simulink model "hopping_daisy"  (R2026b)
settings: Solver=FixedStepDiscrete  StartTime=0  StopTime=10  FixedStep=1
values from neighbouring files (symbols this model uses):
  daisy_bitmap = <binary blob, 10705 chars, not shown>    [hopping_daisy_dd.sldd]
  DAISY_HEIGHT = 40.0    [hopping_daisy_dd.sldd]
  DAISY_WIDTH = 40.0    [hopping_daisy_dd.sldd]
  DAISY_X_START = 80.0    [hopping_daisy_dd.sldd]
  GAME_INIT = 1.0    [hopping_daisy_dd.sldd]
  GAME_STARTED = 2.0    [hopping_daisy_dd.sldd]
  GAME_STOPPED = 3.0    [hopping_daisy_dd.sldd]
  GROUND_BLUE = 64.0    [hopping_daisy_dd.sldd]
  GROUND_GREEN = 176.0    [hopping_daisy_dd.sldd]
  GROUND_RED = 48.0    [hopping_daisy_dd.sldd]
  GROUND_Y_START = 400.0    [hopping_daisy_dd.sldd]
  H_SYNC_END = 752.0    [hopping_daisy_dd.sldd]
  H_SYNC_START = 656.0    [hopping_daisy_dd.sldd]
  H_TOTAL = 800.0    [hopping_daisy_dd.sldd]
  H_VISIBLE = 640.0    [hopping_daisy_dd.sldd]
  obstacle_bitmap = <binary blob, 6837 chars, not shown>    [hopping_daisy_dd.sldd]
  OBSTACLE_HEIGHT = 40.0    [hopping_daisy_dd.sldd]
  OBSTACLE_WIDTH = 20.0    [hopping_daisy_dd.sldd]
  OBSTACLE_Y_START = 360.0    [hopping_daisy_dd.sldd]
  SKY_BLUE = 255.0    [hopping_daisy_dd.sldd]
  SKY_GREEN = 128.0    [hopping_daisy_dd.sldd]
  SKY_RED = 0.0    [hopping_daisy_dd.sldd]
  SYNC_N_DEFAULT = 0.0    [hopping_daisy_dd.sldd]
  V_SYNC_END = 492.0    [hopping_daisy_dd.sldd]
  V_SYNC_START = 490.0    [hopping_daisy_dd.sldd]
  V_TOTAL = 525.0    [hopping_daisy_dd.sldd]
  V_VISIBLE = 480.0    [hopping_daisy_dd.sldd]
libraries: hdlsllib x29, simulink x2
settings Model: DataDictionary=hopping_daisy_dd.sldd  Creator=guion  LastModifiedBy=guion
settings OptimizationCC: BlockReduction=off  ConditionallyExecuteInputs=off  DefaultParameterBehavior=Inlined
settings DebuggingCC: SingleTaskRateTransMsg=error

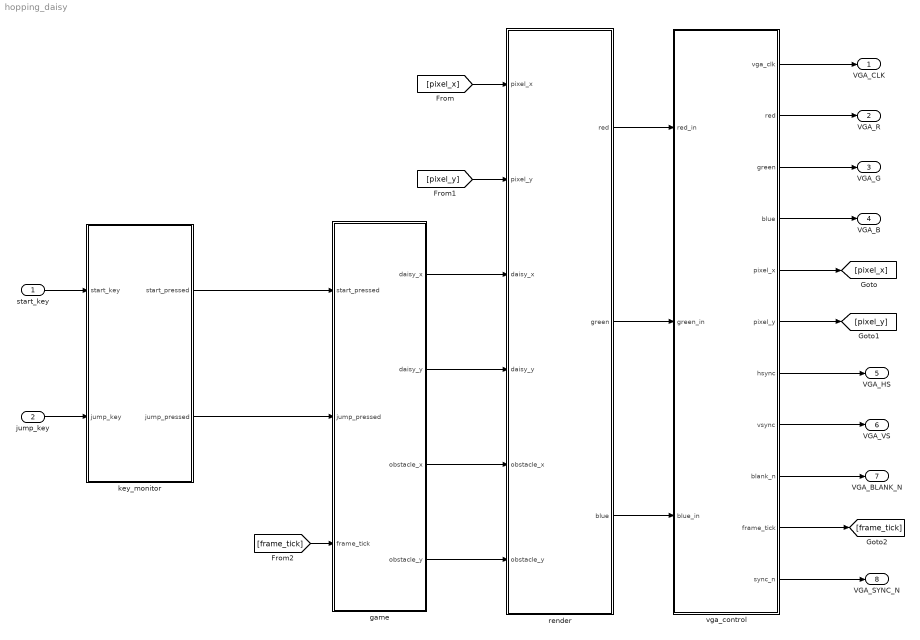
== system hopping_daisy ==
  start_key : Inport  OutDataTypeStr=boolean
  jump_key : Inport  Port=2  OutDataTypeStr=boolean
  game : Subsystem
  key_monitor : Subsystem
  render : Subsystem
  vga_control : Subsystem
  VGA_CLK : Outport
  VGA_R : Outport  Port=2
  VGA_G : Outport  Port=3
  VGA_B : Outport  Port=4
  VGA_HS : Outport  Port=5
  VGA_VS : Outport  Port=6
  VGA_BLANK_N : Outport  Port=7
  VGA_SYNC_N : Outport  Port=8
  wires:
  jump_key/1 -> key_monitor/2(jump_key)
  vga_control/3(green) -> VGA_G/1
  vga_control/9(blank_n) -> VGA_BLANK_N/1
  start_key/1 -> key_monitor/1(start_key)
  vga_control/7(hsync) -> VGA_HS/1
  vga_control/8(vsync) -> VGA_VS/1
  vga_control/2(red) -> VGA_R/1
  vga_control/11(sync_n) -> VGA_SYNC_N/1
  vga_control/4(blue) -> VGA_B/1
  vga_control/1(vga_clk) -> VGA_CLK/1
  key_monitor/1(start_pressed) -> game/1(start_pressed)
  vga_control/5(pixel_x) -> [pixel_x]
  vga_control/6(pixel_y) -> [pixel_y]
  key_monitor/2(jump_pressed) -> game/2(jump_pressed)
  render/1(red) -> vga_control/1(red_in)
  render/2(green) -> vga_control/2(green_in)
  render/3(blue) -> vga_control/3(blue_in)
  vga_control/10(frame_tick) -> [frame_tick]
  [frame_tick] -> game/3(frame_tick)
  [pixel_x] -> render/1(pixel_x)
  [pixel_y] -> render/2(pixel_y)
  game/3(obstacle_x) -> render/5(obstacle_x)
  game/4(obstacle_y) -> render/6(obstacle_y)
  game/2(daisy_y) -> render/4(daisy_y)
  game/1(daisy_x) -> render/3(daisy_x)

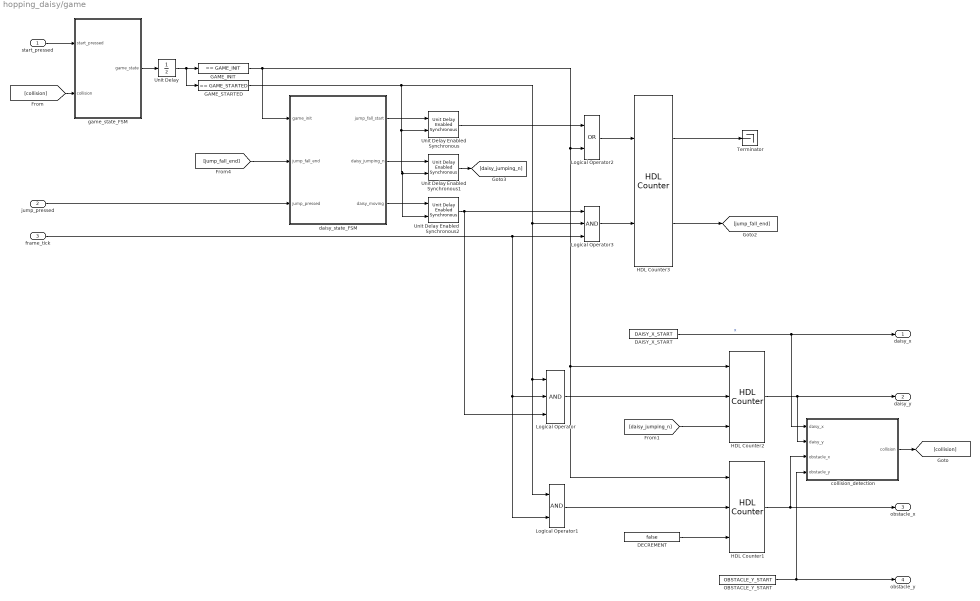
== system hopping_daisy/game ==
  start_pressed : Inport
  jump_pressed : Inport  Port=2
  frame_tick : Inport  Port=3
  DAISY_X_START : Constant  Value=DAISY_X_START  SampleTime=1
  DECREMENT : Constant  Value=false  SampleTime=1
  GAME_INIT : hdlsllib/Logic and Bit Operations/Compare To Constant  relop===  const=GAME_INIT  OutDataTypeStr=boolean
  GAME_STARTED : hdlsllib/Logic and Bit Operations/Compare To Constant  relop===  const=GAME_STARTED  OutDataTypeStr=boolean
  HDL Counter1 : hdlsllib/Sources/HDL Counter  CountType=Count limited  CountInit=OBSTACLE_X_START  CountStep=OBSTACLE_X_SPEED  CountMax=0  CountFromType=Initial value  CountFrom=OBSTACLE_X_START  CountResetPort=on  CountLoadPort=off  CountEnbPort=on  CountDirPort=on  CountHitOutputPort=off  CountDataType=Unsigned  CountWordLen=10  CountFracLen=0  CountSampTime=1
  HDL Counter2 : hdlsllib/Sources/HDL Counter  CountType=Free running  CountInit=DAISY_Y_START  CountStep=DAISY_Y_SPEED  CountMax=0  CountFromType=Initial value  CountFrom=DAISY_Y_START  CountResetPort=on  CountLoadPort=off  CountEnbPort=on  CountDirPort=on  CountHitOutputPort=off  CountDataType=Unsigned  CountWordLen=10  CountFracLen=0  CountSampTime=1
  HDL Counter3 : hdlsllib/Sources/HDL Counter  CountType=Count limited  CountInit=0  CountStep=1  CountMax=DAISY_JUMP_TIMER  CountFromType=Initial value  CountFrom=0  CountResetPort=on  CountLoadPort=off  CountEnbPort=on  CountDirPort=off  CountHitOutputPort=on  CountDataType=Unsigned  CountWordLen=8  CountFracLen=0  CountSampTime=1
  Logical Operator : Logic  Inputs=3  AllPortsSameDT=off  OutDataTypeStr=boolean
  Logical Operator1 : Logic  AllPortsSameDT=off  OutDataTypeStr=boolean
  Logical Operator2 : Logic  Operator=OR  AllPortsSameDT=off  OutDataTypeStr=boolean
  Logical Operator3 : Logic  Inputs=3  AllPortsSameDT=off  OutDataTypeStr=boolean
  OBSTACLE_Y_START : Constant  Value=OBSTACLE_Y_START  SampleTime=1
  Terminator : Terminator
  Unit Delay : UnitDelay  SampleTime=-1
  Unit Delay Enabled Synchronous : hdlsllib/Discrete/Unit Delay Enabled Synchronous  InitialCondition=0  SampleTime=-1
  Unit Delay Enabled Synchronous1 : hdlsllib/Discrete/Unit Delay Enabled Synchronous  InitialCondition=0  SampleTime=-1
  Unit Delay Enabled Synchronous2 : hdlsllib/Discrete/Unit Delay Enabled Synchronous  InitialCondition=0  SampleTime=-1
  collision_detection : Stateflow chart  TreatAsAtomicUnit=on
  daisy_state_FSM : Stateflow chart  TreatAsAtomicUnit=on
      settings: PortSchema="{\"entries\":[{\"content\":{\"sides\":[{\"content\":{\"connectorIds\":[\"In3\",\"In2\",\"In1\"]},\"type\":\"ConnectorPlacement.EquallySpacedRectSide\",\"uuid\":\"e380e228-78e2-4647-af80-acffbeffbf1f\"},{\"content\":{\"connectorIds\":[\"Out1\",\"Out2\",\"Out3\"],\"side\":\"RIGHT\"},\"type\":\"ConnectorPlacement.EquallySpacedRectSide\",\"uuid\":\"b21a9855-612f-46de-ac94-f0d80908291b\"},{\"content\":{\"side\":\"TOP\"},\"type\":\"ConnectorPlacement.EquallySpacedRectSide\",\"uuid\":\"886d6f19-6a3a-4b5a-8f9c-848e91066fef\"}]},\"type\":\"ConnectorPlacement.EquallySpacedConnector\",\"uuid\":\"50e48c1d-c53f-469b-b40b-f4959e901b9a\"}],\"packageUris\":[\"http://schema.mathworks.com/mf0/Connector/R2020b\"],\"version\":\"1.0\"}"
  game_state_FSM : Stateflow chart  TreatAsAtomicUnit=on
  daisy_x : Outport
  daisy_y : Outport  Port=2
  obstacle_x : Outport  Port=3
  obstacle_y : Outport  Port=4
  wires:
  start_pressed/1 -> game_state_FSM/1(start_pressed)
  game_state_FSM/1(game_state) -> Unit Delay/1
  jump_pressed/1 -> daisy_state_FSM/1(jump_pressed)
  Logical Operator/1 -> HDL Counter2/2
  DAISY_X_START/1 -> collision_detection/1(daisy_x), daisy_x/1  "x"
  DECREMENT/1 -> HDL Counter1/3
  HDL Counter2/1 -> collision_detection/2(daisy_y), daisy_y/1
  Unit Delay/1 -> GAME_INIT/1, GAME_STARTED/1
  GAME_INIT/1 -> daisy_state_FSM/3(game_init), Logical Operator2/2, HDL Counter2/1, HDL Counter1/1
  GAME_STARTED/1 -> Unit Delay Enabled Synchronous2/2, Unit Delay Enabled Synchronous1/2, Unit Delay Enabled Synchronous/2, Logical Operator3/2, Logical Operator/1, Logical Operator1/1
  Logical Operator1/1 -> HDL Counter1/2
  HDL Counter3/2 -> [jump_fall_end]
  [jump_fall_end] -> daisy_state_FSM/2(jump_fall_end)
  Logical Operator2/1 -> HDL Counter3/1
  Logical Operator3/1 -> HDL Counter3/2
  daisy_state_FSM/1(jump_fall_start) -> Unit Delay Enabled Synchronous/1
  Unit Delay Enabled Synchronous1/1 -> [daisy_jumping_n]
  daisy_state_FSM/2(daisy_jumping_n) -> Unit Delay Enabled Synchronous1/1
  Unit Delay Enabled Synchronous/1 -> Logical Operator2/1
  frame_tick/1 -> Logical Operator1/2, Logical Operator/2, Logical Operator3/3
  [daisy_jumping_n] -> HDL Counter2/3
  Unit Delay Enabled Synchronous2/1 -> Logical Operator/3, Logical Operator3/1
  daisy_state_FSM/3(daisy_moving) -> Unit Delay Enabled Synchronous2/1
  HDL Counter3/1 -> Terminator/1
  OBSTACLE_Y_START/1 -> collision_detection/4(obstacle_y), obstacle_y/1
  HDL Counter1/1 -> obstacle_x/1, collision_detection/3(obstacle_x)
  collision_detection/1(collision) -> [collision]
  [collision] -> game_state_FSM/2(collision)

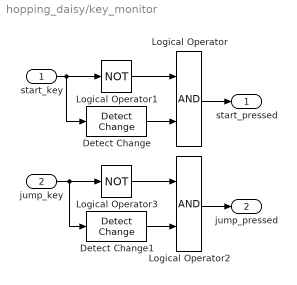
== system hopping_daisy/key_monitor ==
  start_key : Inport
  jump_key : Inport  Port=2
  Detect Change : simulink/Logic and Bit Operations/Detect Change  vinit=0  OutDataTypeStr=boolean
      settings: LibrarySourceBlock=|
      | hdlsllib/Logic and Bit
      | Operations/Detect
      | Change
  Detect Change1 : simulink/Logic and Bit Operations/Detect Change  vinit=0  OutDataTypeStr=boolean
      settings: LibrarySourceBlock=|
      | hdlsllib/Logic and Bit
      | Operations/Detect
      | Change
  Logical Operator : Logic  AllPortsSameDT=off  OutDataTypeStr=boolean
  Logical Operator1 : Logic  Operator=NOT  AllPortsSameDT=off  OutDataTypeStr=boolean
  Logical Operator2 : Logic  AllPortsSameDT=off  OutDataTypeStr=boolean
  Logical Operator3 : Logic  Operator=NOT  AllPortsSameDT=off  OutDataTypeStr=boolean
  start_pressed : Outport
  jump_pressed : Outport  Port=2
  wires:
  Logical Operator/1 -> start_pressed/1
  start_key/1 -> Logical Operator1/1, Detect Change/1
  Logical Operator1/1 -> Logical Operator/1
  Detect Change/1 -> Logical Operator/2
  Logical Operator2/1 -> jump_pressed/1
  Detect Change1/1 -> Logical Operator2/2
  Logical Operator3/1 -> Logical Operator2/1
  jump_key/1 -> Detect Change1/1, Logical Operator3/1

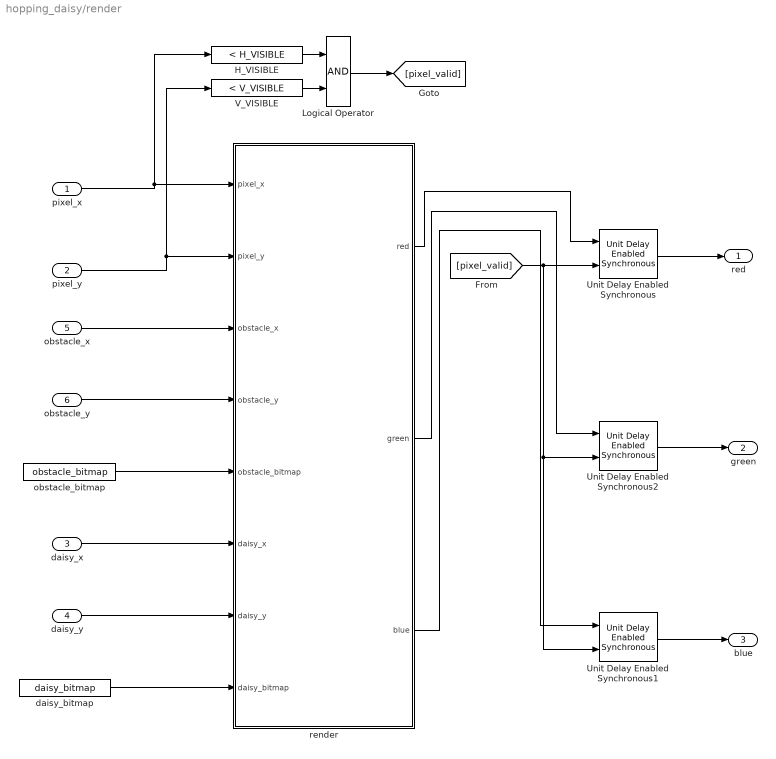
== system hopping_daisy/render ==
  pixel_x : Inport
  pixel_y : Inport  Port=2
  daisy_x : Inport  Port=3
  daisy_y : Inport  Port=4
  obstacle_x : Inport  Port=5
  obstacle_y : Inport  Port=6
  H_VISIBLE : hdlsllib/Logic and Bit Operations/Compare To Constant  relop=<  const=H_VISIBLE  OutDataTypeStr=boolean
  Logical Operator : Logic  AllPortsSameDT=off  OutDataTypeStr=boolean
  Unit Delay Enabled Synchronous : hdlsllib/Discrete/Unit Delay Enabled Synchronous  InitialCondition=0.0  SampleTime=-1
  Unit Delay Enabled Synchronous1 : hdlsllib/Discrete/Unit Delay Enabled Synchronous  InitialCondition=0.0  SampleTime=-1
  Unit Delay Enabled Synchronous2 : hdlsllib/Discrete/Unit Delay Enabled Synchronous  InitialCondition=0.0  SampleTime=-1
  V_VISIBLE : hdlsllib/Logic and Bit Operations/Compare To Constant  relop=<  const=V_VISIBLE  OutDataTypeStr=boolean
  daisy_bitmap : Constant  Value=daisy_bitmap  SampleTime=1
  obstacle_bitmap : Constant  Value=obstacle_bitmap  SampleTime=1
  render : Stateflow chart  TreatAsAtomicUnit=on
  red : Outport
  green : Outport  Port=2
  blue : Outport  Port=3
  wires:
  Unit Delay Enabled Synchronous/1 -> red/1
  Unit Delay Enabled Synchronous2/1 -> green/1
  Unit Delay Enabled Synchronous1/1 -> blue/1
  render/3(blue) -> Unit Delay Enabled Synchronous1/1
  render/1(red) -> Unit Delay Enabled Synchronous/1
  render/2(green) -> Unit Delay Enabled Synchronous2/1
  obstacle_x/1 -> render/3(obstacle_x)
  obstacle_y/1 -> render/4(obstacle_y)
  pixel_y/1 -> render/2(pixel_y), V_VISIBLE/1
  pixel_x/1 -> H_VISIBLE/1, render/1(pixel_x)
  Logical Operator/1 -> [pixel_valid]
  H_VISIBLE/1 -> Logical Operator/1
  V_VISIBLE/1 -> Logical Operator/2
  [pixel_valid] -> Unit Delay Enabled Synchronous2/2, Unit Delay Enabled Synchronous1/2, Unit Delay Enabled Synchronous/2
  daisy_x/1 -> render/6(daisy_x)
  daisy_y/1 -> render/7(daisy_y)
  obstacle_bitmap/1 -> render/5(obstacle_bitmap)
  daisy_bitmap/1 -> render/8(daisy_bitmap)

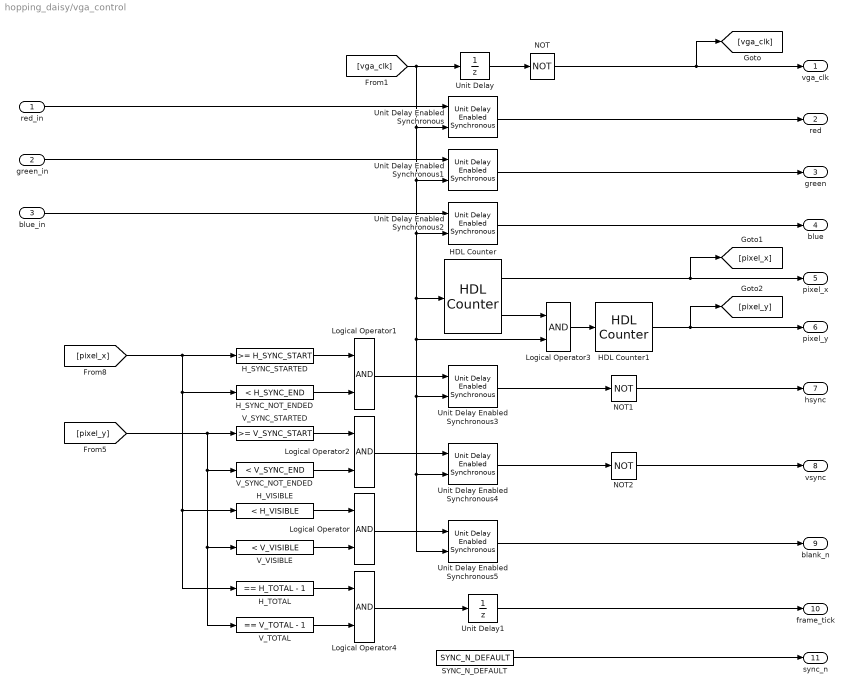
== system hopping_daisy/vga_control ==
  red_in : Inport
  green_in : Inport  Port=2
  blue_in : Inport  Port=3
  HDL Counter : hdlsllib/Sources/HDL Counter  CountType=Count limited  CountInit=0  CountStep=1  CountMax=H_TOTAL - 1  CountFromType=Initial value  CountFrom=0  CountResetPort=off  CountLoadPort=off  CountEnbPort=on  CountDirPort=off  CountHitOutputPort=on  CountDataType=Unsigned  CountWordLen=10  CountFracLen=0  CountSampTime=1
  HDL Counter1 : hdlsllib/Sources/HDL Counter  CountType=Count limited  CountInit=0  CountStep=1  CountMax=V_TOTAL - 1  CountFromType=Initial value  CountFrom=0  CountResetPort=off  CountLoadPort=off  CountEnbPort=on  CountDirPort=off  CountHitOutputPort=off  CountDataType=Unsigned  CountWordLen=10  CountFracLen=0  CountSampTime=1
  H_SYNC_NOT_ENDED : hdlsllib/Logic and Bit Operations/Compare To Constant  relop=<  const=H_SYNC_END  OutDataTypeStr=boolean
  H_SYNC_STARTED : hdlsllib/Logic and Bit Operations/Compare To Constant  relop=>=  const=H_SYNC_START  OutDataTypeStr=boolean
  H_TOTAL : hdlsllib/Logic and Bit Operations/Compare To Constant  relop===  const=H_TOTAL - 1  OutDataTypeStr=boolean
  H_VISIBLE : hdlsllib/Logic and Bit Operations/Compare To Constant  relop=<  const=H_VISIBLE  OutDataTypeStr=boolean
  Logical Operator{,1..4} (5 alike) : Logic  AllPortsSameDT=off  OutDataTypeStr=boolean
  NOT : Logic  Operator=NOT  IconShape=distinctive  AllPortsSameDT=off  OutDataTypeStr=boolean
  NOT1 : Logic  Operator=NOT  IconShape=distinctive  AllPortsSameDT=off  OutDataTypeStr=boolean
  NOT2 : Logic  Operator=NOT  IconShape=distinctive  AllPortsSameDT=off  OutDataTypeStr=boolean
  SYNC_N_DEFAULT : Constant  Value=SYNC_N_DEFAULT  SampleTime=1
  Unit Delay : UnitDelay  SampleTime=-1
  Unit Delay Enabled Synchronous{,1..5} (6 alike) : hdlsllib/Discrete/Unit Delay Enabled Synchronous  InitialCondition=0  SampleTime=-1
  Unit Delay1 : UnitDelay  SampleTime=-1
  V_SYNC_NOT_ENDED : hdlsllib/Logic and Bit Operations/Compare To Constant  relop=<  const=V_SYNC_END  OutDataTypeStr=boolean
  V_SYNC_STARTED : hdlsllib/Logic and Bit Operations/Compare To Constant  relop=>=  const=V_SYNC_START  OutDataTypeStr=boolean
  V_TOTAL : hdlsllib/Logic and Bit Operations/Compare To Constant  relop===  const=V_TOTAL - 1  OutDataTypeStr=boolean
  V_VISIBLE : hdlsllib/Logic and Bit Operations/Compare To Constant  relop=<  const=V_VISIBLE  OutDataTypeStr=boolean
  vga_clk : Outport
  red : Outport  Port=2
  green : Outport  Port=3
  blue : Outport  Port=4
  pixel_x : Outport  Port=5
  pixel_y : Outport  Port=6
  hsync : Outport  Port=7
  vsync : Outport  Port=8
  blank_n : Outport  Port=9
  frame_tick : Outport  Port=10
  sync_n : Outport  Port=11
  wires:
  H_SYNC_STARTED/1 -> Logical Operator1/1
  Unit Delay/1 -> NOT/1
  [pixel_x] -> H_SYNC_STARTED/1, H_SYNC_NOT_ENDED/1, H_TOTAL/1, H_VISIBLE/1
  V_SYNC_STARTED/1 -> Logical Operator2/1
  V_VISIBLE/1 -> Logical Operator/2
  [pixel_y] -> V_TOTAL/1, V_VISIBLE/1, V_SYNC_NOT_ENDED/1, V_SYNC_STARTED/1
  SYNC_N_DEFAULT/1 -> sync_n/1
  [vga_clk] -> Unit Delay/1, Unit Delay Enabled Synchronous1/2, Unit Delay Enabled Synchronous5/2, Unit Delay Enabled Synchronous4/2, Unit Delay Enabled Synchronous3/2, Logical Operator3/2, HDL Counter/1, Unit Delay Enabled Synchronous2/2, Unit Delay Enabled Synchronous/2
  H_VISIBLE/1 -> Logical Operator/1
  H_SYNC_NOT_ENDED/1 -> Logical Operator1/2
  V_SYNC_NOT_ENDED/1 -> Logical Operator2/2
  NOT2/1 -> vsync/1
  NOT1/1 -> hsync/1
  red_in/1 -> Unit Delay Enabled Synchronous/1
  Unit Delay Enabled Synchronous/1 -> red/1
  Unit Delay Enabled Synchronous2/1 -> blue/1
  Unit Delay Enabled Synchronous1/1 -> green/1
  green_in/1 -> Unit Delay Enabled Synchronous1/1
  blue_in/1 -> Unit Delay Enabled Synchronous2/1
  HDL Counter/1 -> [pixel_x], pixel_x/1
  HDL Counter1/1 -> [pixel_y], pixel_y/1
  Logical Operator1/1 -> Unit Delay Enabled Synchronous3/1
  Unit Delay Enabled Synchronous4/1 -> NOT2/1
  Logical Operator2/1 -> Unit Delay Enabled Synchronous4/1
  Unit Delay Enabled Synchronous5/1 -> blank_n/1
  Logical Operator/1 -> Unit Delay Enabled Synchronous5/1
  Logical Operator3/1 -> HDL Counter1/1
  HDL Counter/2 -> Logical Operator3/1
  NOT/1 -> [vga_clk], vga_clk/1
  Unit Delay Enabled Synchronous3/1 -> NOT1/1
  Unit Delay1/1 -> frame_tick/1
  Logical Operator4/1 -> Unit Delay1/1
  H_TOTAL/1 -> Logical Operator4/1
  V_TOTAL/1 -> Logical Operator4/2

== stateflow chart hopping_daisy/game/game_state_FSM ==
  state INIT
  state STARTED
  state STOPPED
  (default) -> INIT
  INIT -> STARTED : [start_pressed]{game_state = GAME_STARTED;}
  STOPPED -> INIT : [start_pressed]{game_state = GAME_INIT;}
  STARTED -> STOPPED : [start_pressed || collision]{game_state = GAME_STOPPED;}
  data: start_pressed input; game_state output; GAME_INIT parameter; GAME_STARTED parameter; GAME_STOPPED parameter; collision input

== stateflow chart hopping_daisy/render/render ==
  (default) -> (junction 140) : {red = SKY_RED;
      | green = SKY_GREEN;
      | blue = SKY_BLUE;}
  (default) -> (junction 108) [commented out]
  (junction 140) -> (junction 145) [order 1] : [pixel_y >= GROUND_Y_START]
  (junction 140) -> (junction 161) [order 2]
  (junction 145) -> (junction 143) : {red = GROUND_RED;
      | green = GROUND_GREEN;
      | blue = GROUND_BLUE;}
  (junction 108) -> (junction 110) [commented out] : [(pixel_x >= daisy_x) && (pixel_x < (daisy_x + DAISY_WIDTH)) && (pixel_y >= daisy_y) && (pixel_y < (daisy_y + DAISY_HEIGHT))]
  (junction 108) -> (junction 73) [commented out]
  (junction 110) -> (junction 112) [commented out] : {red = OBSTACLE_RED;
      | green = OBSTACLE_GREEN;
      | blue = OBSTACLE_BLUE;}
  (junction 143) -> (junction 161)
  (junction 73) -> (junction 74) [commented out] : [(pixel_x >= obstacle_x) && (pixel_x < (obstacle_x + OBSTACLE_WIDTH)) && (pixel_y >= obstacle_y) && (pixel_y < (obstacle_y + OBSTACLE_HEIGHT))]
  (junction 73) -> (junction 75) [commented out]
  (junction 161) -> (junction 164)
  (junction 74) -> (junction 79) [commented out] : {red = get_red(pixel_x, pixel_y, obstacle_x, obstacle_y);
      | green = get_green(pixel_x, pixel_y, obstacle_x, obstacle_y);
      | blue = get_blue(pixel_x, pixel_y, obstacle_x, obstacle_y);}
  (junction 164) -> (junction 166) [order 1] : [(pixel_x >= obstacle_x) && (pixel_x < (obstacle_x + OBSTACLE_WIDTH)) && (pixel_y >= obstacle_y) && (pixel_y < (obstacle_y + OBSTACLE_HEIGHT))]
  (junction 75) -> (junction 76) [commented out] : [pixel_y >= GROUND_Y_START]
  (junction 164) -> (junction 180) [order 2]
  (junction 166) -> (junction 175) : [~get_transparent(pixel_x, pixel_y, obstacle_x, obstacle_y, obstacle_bitmap)]{
      | red = get_red(pixel_x, pixel_y, obstacle_x, obstacle_y, obstacle_bitmap);
      | green = get_green(pixel_x, pixel_y, obstacle_x, obstacle_y, obstacle_bitmap);
      | blue = get_blue(pixel_x, pixel_y, obstacle_x, obstacle_y, obstacle_bitmap);}
  (junction 75) -> (junction 77) [commented out] : {red = SKY_RED;
      | green = SKY_GREEN;
      | blue = SKY_BLUE;}
  (junction 76) -> (junction 78) [commented out] : {red = GROUND_RED;
      | green = GROUND_GREEN;
      | blue = GROUND_BLUE;}
  (junction 175) -> (junction 180)
  (junction 180) -> (junction 184)
  (junction 78) -> (junction 77) [commented out]
  (junction 79) -> (junction 78) [commented out]
  (junction 112) -> (junction 79) [commented out]
  (junction 77) -> (junction 80) [commented out]
  (junction 184) -> (junction 186) [order 1] : [(pixel_x >= daisy_x) && (pixel_x < (daisy_x + DAISY_WIDTH)) && (pixel_y >= daisy_y) && (pixel_y < (daisy_y + DAISY_HEIGHT))]
  (junction 186) -> (junction 188) : [~get_transparent(pixel_x, pixel_y, daisy_x, daisy_y, daisy_bitmap)]{
      | red = get_red(pixel_x, pixel_y, daisy_x, daisy_y, daisy_bitmap);
      | green = get_green(pixel_x, pixel_y, daisy_x, daisy_y, daisy_bitmap);
      | blue = get_blue(pixel_x, pixel_y, daisy_x, daisy_y, daisy_bitmap);}
  (junction 184) -> (junction 146) [order 2]
  (junction 188) -> (junction 146)
  (junction 146) -> (junction 192)
  data: x function_input; y function_input; objx function_input; objy function_input; ret function_output; bitmap function_input; x function_input; y function_input; objx function_input; objy function_input; ret function_output; bitmap function_input; x function_input; y function_input; objx function_input; objy function_input; ret function_output; bitmap function_input; x function_input; y function_input; objx function_input; objy function_input; ret function_output; bitmap function_input; red output; pixel_x input; pixel_y input; OBSTACLE_WIDTH parameter; SKY_RED parameter; SKY_GREEN parameter; SKY_BLUE parameter; GROUND_RED parameter; GROUND_GREEN parameter; GROUND_BLUE parameter; green output; blue output; obstacle_x input; obstacle_y input; obstacle_bitmap input; OBSTACLE_HEIGHT parameter; GROUND_Y_START parameter; daisy_x input; daisy_y input; DAISY_HEIGHT parameter; DAISY_WIDTH parameter; daisy_bitmap input
  function ret = get_red(x, y, objx, objy, bitmap):
    | function ret = get_red(x, y, objx, objy, bitmap)
    | %#codegen
    | 
    | % Local sprite coordinates.
    | row = uint16(int16(y) - int16(objy)) + uint16(1);
    | col = uint16(int16(x) - int16(objx)) + uint16(1);
    | 
    | % Extract red from 0xAARRGGBB.
    | pixel = bitmap(row, col);
    | ret = uint8(bitand(bitshift(pixel, -16), uint32(255)));
    | end
  function ret = get_green(x, y, objx, objy, bitmap):
    | function ret = get_green(x, y, objx, objy, bitmap)
    | %#codegen
    | 
    | % Local sprite coordinates.
    | row = uint16(int16(y) - int16(objy)) + uint16(1);
    | col = uint16(int16(x) - int16(objx)) + uint16(1);
    | 
    | % Extract green from 0xAARRGGBB.
    | pixel = bitmap(row, col);
    | ret = uint8(bitand(bitshift(pixel, -8), uint32(255)));
    | end
  function ret = get_blue(x, y, objx, objy, bitmap):
    | function ret = get_blue(x, y, objx, objy, bitmap)
    | %#codegen
    | 
    | % Local sprite coordinates.
    | row = uint16(int16(y) - int16(objy)) + uint16(1);
    | col = uint16(int16(x) - int16(objx)) + uint16(1);
    | 
    | % Extract blue from 0xAARRGGBB.
    | pixel = bitmap(row, col);
    | ret = uint8(bitand(pixel, uint32(255)));
    | end
  function ret = get_transparent(x, y, objx, objy, bitmap):
    | function ret = get_transparent(x, y, objx, objy, bitmap)
    | %#codegen
    | 
    | % Local sprite coordinates.
    | row = uint16(int16(y) - int16(objy)) + uint16(1);
    | col = uint16(int16(x) - int16(objx)) + uint16(1);
    | 
    | % A zero alpha value means fully transparent.
    | pixel = bitmap(row, col);
    | ret = bitshift(pixel, -24) == uint32(0);
    | end

== stateflow chart hopping_daisy/game/daisy_state_FSM ==
  state STANDING
    jump_fall_start = false;
    daisy_jumping_n = true;
    daisy_moving = false;
  state JUMPING
    en:
    jump_fall_start = true;
    daisy_jumping_n = false;
    daisy_moving = true;
    during:
    jump_fall_start = false;
  state FALLING
    en:
    jump_fall_start = true;
    daisy_jumping_n = true;
    daisy_moving = true;
    during:
    jump_fall_start = false;
  (default) -> STANDING
  FALLING -> STANDING [order 2] : [jump_fall_end]
  (junction 28) -> STANDING : [game_init]
  STANDING -> JUMPING : [jump_pressed]
  JUMPING -> (junction 28) [order 1]
  FALLING -> (junction 28) [order 1]
  JUMPING -> FALLING [order 2] : [jump_fall_end]
  data: jump_pressed input; jump_fall_start output; jump_fall_end input; daisy_jumping_n output; game_init input; daisy_moving output

== stateflow chart hopping_daisy/game/collision_detection ==
  (default) -> (junction 37)
  (junction 37) -> (junction 38) [order 1] : [((daisy_y + DAISY_HEIGHT) > obstacle_y) && ...
      |  (daisy_y < (obstacle_y + OBSTACLE_HEIGHT)) && ...
      |  ((daisy_x + DAISY_WIDTH) > obstacle_x) && ...
      |  (daisy_x < (obstacle_x + OBSTACLE_WIDTH))]
  (junction 37) -> (junction 41) [order 2] : {collision = false;}
  (junction 38) -> (junction 43) : {collision = true;}
  (junction 43) -> (junction 41)
  (junction 41) -> (junction 46)
  data: daisy_x input; daisy_y input; obstacle_x input; collision output; OBSTACLE_HEIGHT parameter; DAISY_WIDTH parameter; obstacle_y input; OBSTACLE_WIDTH parameter; DAISY_HEIGHT parameter
